simulink model "MSFcascade"  (Simulink 10.2)
settings: Solver=ode8  StartTime=0.0  StopTime=inf  FixedStep=100e-3  MaxStep=5  RelTol=1e-6  AbsTol=1e-6
StopFcn:
  | msfplot
libraries: slrealtimeutilitieslib x2, dspnetwork x2, simulink_need_slupdate x2
settings Model: Creator=Prashant  LastModifiedBy=Prashant  ModifiedComment=Prashant -- Wed Sep 30 22:08:04 2020 -- Version 8.300000e+00  ExtModeTrigMode=oneshot  ExtModeArmWhenConnect=off
settings Model: ModifiedHistory=|
  | Prashant -- Wed Sep 30 22:08:04 2020 -- Version 8.300000e+00
  | 
  | Prashant -- Tue Sep 29 12:44:36 2020 -- Version 8.200000e+00
settings SolverCC: AutoScaleAbsTol=off
settings DataIOCC: SaveOutput=off  SaveState=on
settings OptimizationCC: BlockReduction=off  BooleanDataType=off
settings DebuggingCC: SignalInfNanChecking=warning  SaveWithParameterizedLinksMsg=none  SignalResolutionControl=TryResolveAllWithWarning  MultiTaskDSMMsg=warning  MultiTaskCondExecSysMsg=none  FcnCallInpInsideContextMsg=error
settings HardwareCC: TargetUnknown=on

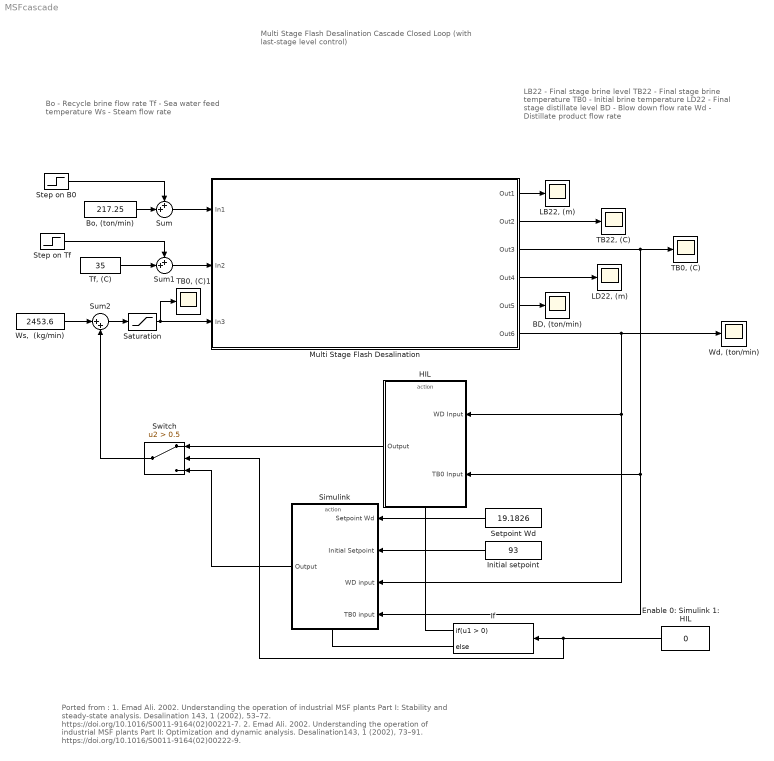
== system MSFcascade ==
  note: Multi Stage Flash Desalination
      | Cascade Closed Loop
      | (with last-stage level control)
  note: Ported from :
      |
      | 1. Emad Ali. 2002. Understanding the operation of industrial MSF plants Part I: Stability and steady-state analysis. Desalination 143, 1 (2002), 53–72. https://doi.org/10.1016/S0011-9164(02)00221-7.
      | 2. Emad Ali. 2002. Understanding the operation of industrial MSF plants Part II: Optimization and dynamic analysis. Desalination143, 1 (2002), 73–91. https://doi.org/10.1016/S0011-9164(02)00222-9.
  note: Bo - Recycle brine flow rate
      | Tf - Sea water feed temperature
      | Ws - Steam flow rate
  note: LB22 - Final stage brine level
      | TB22 - Final stage brine temperature
      | TB0 - Initial brine temperature
      | LD22 - Final stage distillate level
      | BD - Blow down flow rate
      | Wd - Distillate product flow rate
  "BD, (ton/min)" : Scope
  "Bo, (ton/min)" : Constant  Value=217.25
  "Enable 0: Simulink 1:     HIL     " : Constant  Value=0  OutDataTypeStr=double
  HIL : Subsystem  TreatAsAtomicUnit=on
  If : If
  Initial setpoint : Constant  Value=93
  "LB22, (m)" : Scope
  "LD22, (m)" : Scope
  Multi Stage Flash Desalination : Subsystem  mask(Simple MAsk){fname=x68.inc, Us=49.767, U=35.0, Wf=143.8167, Rej=95.3500, Ts=98.10, Wd=[19.1826  29.2841], LB=[0.556818  -50 0.001], LD=[0.3394 -5 0.01], N=[3 19], v=[0 0 0 0 0 0.0]}
      mask prompts: fname "File name for Initial condition of the states"; Us "Heat transfer coeff. of Brine Heater, kJ/min C m2"; U "Heat transfer coeff. of tube, kJ/min C m2"; Wf "Sea Water feed rate, (ton/hr)"; Rej "Reject flow rate, (ton/hr)"; Ts "Steam Temperature, (C)"; Wd "Initial condition for Distillate product and Blowdown"; LB "Setpoint, proporional gain, integral time  for Brine level control"; LD "Setpoint, proportional gain, integral time for distillate level control"; N "Number of rejection and recovery stages"; v "Noise variance"
      mask help:
      | (1) Insert the file name that contains the initial condition for the states
      |
      | (2) Insert the physical parameter values:
      |
      | Us, U, Wf, Rej, Ts, Wdss Bdss, LBsp, kc1, ki1, LDsp, kc2 ki2, NREJ, NREC
      |
      | For definition and nominal values for the process states and parameters, click on the Help bar
      mask init:
      | param=[Us U Wf Rej Ts Wd LB LD N];
      mask Help: web(['file:///' which('msfdes.htm')])
      mask Display: image(imread('msf.jpg'))
  Saturation : Saturate  UpperLimit=3000  LowerLimit=1000
  Setpoint Wd : Constant  Value=19.1826
  Simulink : Subsystem  TreatAsAtomicUnit=on
  Step on B0 : Step  Time=10  After=0  SampleTime=0
  Step on Tf : Step  Time=10  After=0  SampleTime=0
  Sum : Sum  Inputs=++|  InputSameDT=on  SaturateOnIntegerOverflow=on  OutDataTypeStr=Inherit: Same as first input
  Sum1 : Sum  Inputs=++|  InputSameDT=on  SaturateOnIntegerOverflow=on  OutDataTypeStr=Inherit: Same as first input
  Sum2 : Sum  Inputs=|++  InputSameDT=on  SaturateOnIntegerOverflow=on  OutDataTypeStr=Inherit: Same as first input
  Switch : Switch  Criteria=u2 > Threshold  Threshold=0.5
  "TB0, (C)" : Scope
  "TB0, (C)1" : Scope
  "TB22, (C)" : Scope
  "Tf, (C)" : Constant  Value=35
  "Wd, (ton/min)" : Scope
  "Ws,  (kg/min)" : Constant  Value=2453.6
  wires:
  Multi Stage Flash Desalination/1(Out1) -> "LB22, (m)"/1
  Multi Stage Flash Desalination/2(Out2) -> "TB22, (C)"/1
  Multi Stage Flash Desalination/5(Out5) -> "BD, (ton/min)"/1
  Multi Stage Flash Desalination/4(Out4) -> "LD22, (m)"/1
  Step on Tf/1 -> Sum1/1
  Sum1/1 -> Multi Stage Flash Desalination/2(In2)
  "Tf, (C)"/1 -> Sum1/2
  Step on B0/1 -> Sum/1
  "Bo, (ton/min)"/1 -> Sum/2
  Sum/1 -> Multi Stage Flash Desalination/1(In1)
  Multi Stage Flash Desalination/3(Out3) -> Simulink/4("TB0 input "), HIL/2(TB0 Input), "TB0, (C)"/1
  "Ws,  (kg/min)"/1 -> Sum2/1
  Sum2/1 -> Saturation/1
  Saturation/1 -> Multi Stage Flash Desalination/3(In3), "TB0, (C)1"/1
  Multi Stage Flash Desalination/6(Out6) -> "Wd, (ton/min)"/1, Simulink/3(WD input), HIL/1(WD Input)
  "Enable 0: Simulink 1:     HIL     "/1 -> Switch/2, If/1
  If/1 -> HIL/Action
  If/2 -> Simulink/Action
  Simulink/1(Output) -> Switch/3
  HIL/1(Output) -> Switch/1
  Switch/1 -> Sum2/2
  Initial setpoint/1 -> Simulink/2(Initial Setpoint)
  Setpoint Wd/1 -> Simulink/1(Setpoint Wd)

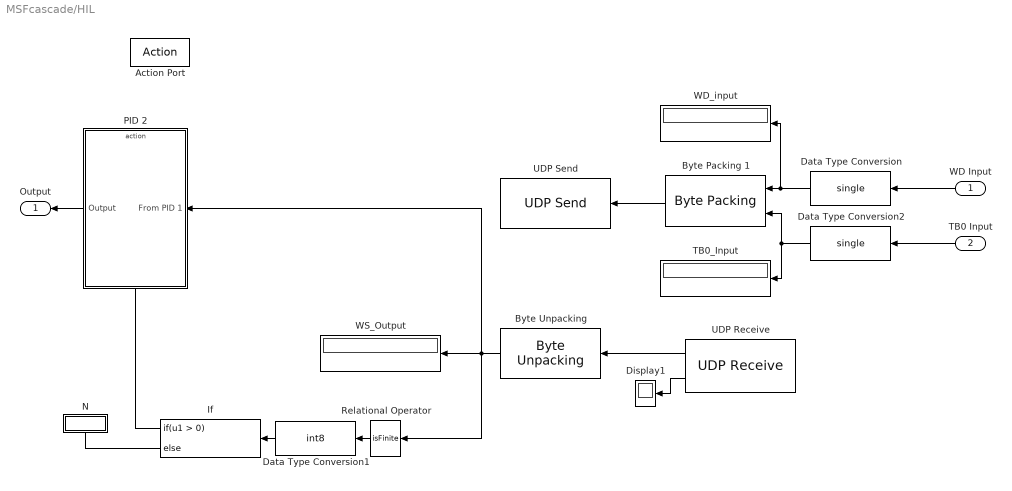
== system MSFcascade/HIL ==
  WD Input : Inport
  TB0 Input : Inport  Port=2
  Action Port : ActionPort  ActionPortLabel=if(u1 > 0)
  Byte Packing 1 : slrealtimeutilitieslib/Byte Packing  MaskPackedDataType=uint8  MaskUnpackedDataTypes={'single','single'}  MaskAlignment=1
  "Byte Unpacking " : slrealtimeutilitieslib/Byte Unpacking  MaskUnpackedDataTypes={'single'}  MaskUnpackedDataSizes={[1]}  MaskAlignment=1
      settings: SourceProductBaseCode=XP
  Data Type Conversion : DataTypeConversion  OutDataTypeStr=single
  Data Type Conversion1 : DataTypeConversion  OutDataTypeStr=int8
  Data Type Conversion2 : DataTypeConversion  OutDataTypeStr=single
  Display1 : Display
  If : If
  N : Subsystem  TreatAsAtomicUnit=on
  PID 2 : Subsystem  TreatAsAtomicUnit=on
  Relational Operator : RelationalOperator  Operator=isFinite  OutDataTypeStr=boolean  RndMeth=Simplest
  TB0_Input : Display
  UDP Receive : dspnetwork/UDP Receive  localURL='0.0.0.0'  localPort=11  remoteURL='127.0.0.1'  remotePort=-1  recvBufferSize=8192  dims=4  signalDatatype=uint8  isComplex=off  isVarSize=off  showBlockingTime=off  blockingTime=0  sampletime=0  blockPlatform=[]
  UDP Send : dspnetwork/UDP Send  remoteURL='127.0.0.1'  remotePort=12  localURL='0.0.0.0'  localPortSource=Automatically determine  localPort=-1  sendBufferSize=8192  sampletime=-1  blockPlatform=[]  separateLengthPort=0
  WD_input : Display
  WS_Output : Display
  Output : Outport  VectorParamsAs1DForOutWhenUnconnected=off
  wires:
  Data Type Conversion/1 -> WD_input/1, Byte Packing 1/1
  Byte Packing 1/1 -> UDP Send/1
  UDP Receive/1 -> "Byte Unpacking "/1
  UDP Receive/2 -> Display1/1
  WD Input/1 -> Data Type Conversion/1
  If/1 -> PID 2/Action
  PID 2/1(Output) -> Output/1
  Data Type Conversion1/1 -> If/1
  Relational Operator/1 -> Data Type Conversion1/1
  If/2 -> N/Action
  "Byte Unpacking "/1 -> PID 2/1(From PID 1), WS_Output/1, Relational Operator/1
  TB0 Input/1 -> Data Type Conversion2/1
  Data Type Conversion2/1 -> TB0_Input/1, Byte Packing 1/2

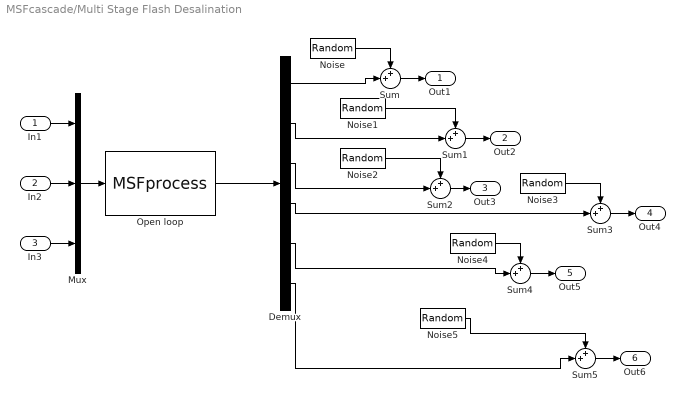
== system MSFcascade/Multi Stage Flash Desalination ==
  In1 : Inport
  In2 : Inport  Port=2
  In3 : Inport  Port=3
  Demux : Demux  Outputs=6
      settings: DisplayOption=none
  Mux : Mux  Inputs=3
  Noise : RandomNumber  Variance=v(1)  SampleTime=0
  Noise1 : RandomNumber  Variance=v(2)  SampleTime=0
  Noise2 : RandomNumber  Variance=v(3)  SampleTime=0
  Noise3 : RandomNumber  Variance=v(4)  SampleTime=0
  Noise4 : RandomNumber  Variance=v(5)  SampleTime=0
  Noise5 : RandomNumber  Variance=v(6)  SampleTime=0
  Open loop : S-Function  FunctionName=MSFprocess  Parameters=param,fname  SFunctionDeploymentMode=off  EnableBusSupport=off
  Sum{,1..5} (6 alike) : Sum  Inputs=++|  InputSameDT=on  SaturateOnIntegerOverflow=on  OutDataTypeStr=Inherit: Same as first input
  Out1 : Outport  VectorParamsAs1DForOutWhenUnconnected=off
  Out2 : Outport  Port=2  VectorParamsAs1DForOutWhenUnconnected=off
  Out3 : Outport  Port=3  VectorParamsAs1DForOutWhenUnconnected=off
  Out4 : Outport  Port=4  VectorParamsAs1DForOutWhenUnconnected=off
  Out5 : Outport  Port=5  VectorParamsAs1DForOutWhenUnconnected=off
  Out6 : Outport  Port=6  VectorParamsAs1DForOutWhenUnconnected=off
  wires:
  Open loop/1 -> Demux/1
  Demux/1 -> Sum/2
  Noise/1 -> Sum/1
  Sum/1 -> Out1/1
  Noise1/1 -> Sum1/1
  Sum1/1 -> Out2/1
  Demux/2 -> Sum1/2
  Noise2/1 -> Sum2/1
  Sum2/1 -> Out3/1
  Demux/3 -> Sum2/2
  Noise3/1 -> Sum3/1
  Sum3/1 -> Out4/1
  Demux/4 -> Sum3/2
  Noise4/1 -> Sum4/1
  Sum4/1 -> Out5/1
  Demux/5 -> Sum4/2
  Noise5/1 -> Sum5/1
  Sum5/1 -> Out6/1
  Demux/6 -> Sum5/2
  Mux/1 -> Open loop/1
  In1/1 -> Mux/1
  In2/1 -> Mux/2
  In3/1 -> Mux/3

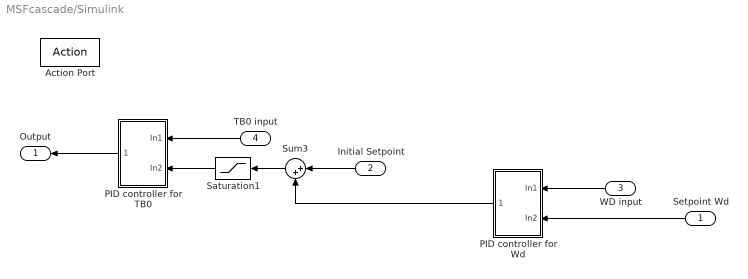
== system MSFcascade/Simulink ==
  Setpoint Wd : Inport
  Initial Setpoint : Inport  Port=2
  WD input : Inport  Port=3
  "TB0 input " : Inport  Port=4
  Action Port : ActionPort  ActionPortLabel=else
  PID controller for TB0 : Subsystem  mask(Simple Mask){P=50, I=10, D=0}
      mask prompts: P "Proportional gain"; I "Integral time"; D "Derivative time"
      mask help: Insert the values of the PID ocntrollers
      mask Help: web(['file:///' which('PID.htm')])
  PID controller for Wd : Subsystem  mask(Simple Mask){P=0.01, I=0.1, D=0}
      mask prompts: P "Proportional gain"; I "Integral time"; D "Derivative time"
      mask help: Insert the values of the PID ocntrollers
      mask Help: web(['file:///' which('PID.htm')])
  Saturation1 : Saturate  UpperLimit=110  LowerLimit=85
  Sum3 : Sum  Inputs=|++  InputSameDT=on  SaturateOnIntegerOverflow=on  OutDataTypeStr=Inherit: Same as first input
  Output : Outport  VectorParamsAs1DForOutWhenUnconnected=off
  wires:
  PID controller for Wd/1(Out1) -> Sum3/2
  Saturation1/1 -> PID controller for TB0/2(In2)
  Sum3/1 -> Saturation1/1
  PID controller for TB0/1(Out1) -> Output/1
  Setpoint Wd/1 -> PID controller for Wd/2(In2)
  WD input/1 -> PID controller for Wd/1(In1)
  "TB0 input "/1 -> PID controller for TB0/1(In1)
  Initial Setpoint/1 -> Sum3/1

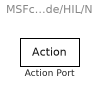
== system MSFcascade/HIL/N ==
  Action Port : ActionPort  ActionPortLabel=else

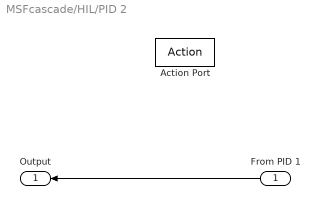
== system MSFcascade/HIL/PID 2 ==
  From PID 1 : Inport
  Action Port : ActionPort  ActionPortLabel=if(u1 > 0)
  Output : Outport  VectorParamsAs1DForOutWhenUnconnected=off
  wires:
  From PID 1/1 -> Output/1

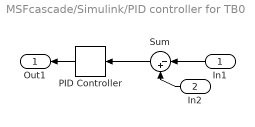
== system MSFcascade/Simulink/PID controller for TB0 ==
  In1 : Inport
  In2 : Inport  Port=2
  PID Controller : simulink_need_slupdate/PID Controller  P=P  I=I  D=D
  Sum : Sum  Inputs=|-+  InputSameDT=on  SaturateOnIntegerOverflow=on  OutDataTypeStr=Inherit: Same as first input
  Out1 : Outport  VectorParamsAs1DForOutWhenUnconnected=off
  wires:
  In1/1 -> Sum/1
  Sum/1 -> PID Controller/1
  PID Controller/1 -> Out1/1
  In2/1 -> Sum/2

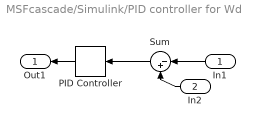
== system MSFcascade/Simulink/PID controller for Wd ==
  In1 : Inport
  In2 : Inport  Port=2
  PID Controller : simulink_need_slupdate/PID Controller  P=P  I=I  D=D
  Sum : Sum  Inputs=|-+  InputSameDT=on  SaturateOnIntegerOverflow=on  OutDataTypeStr=Inherit: Same as first input
  Out1 : Outport  VectorParamsAs1DForOutWhenUnconnected=off
  wires:
  In1/1 -> Sum/1
  Sum/1 -> PID Controller/1
  PID Controller/1 -> Out1/1
  In2/1 -> Sum/2
